simulink model "PSU"  (R2024b)
settings: Solver=VariableStepAuto  StartTime=0.0  StopTime=10.0  RelTol=1e-3
libraries: spsGroundLib x2, spsThreePhaseProgrammableVoltageSourceLib x1, spsThreePhaseBreakerLib x1, spsThreePhaseVIMeasurementLib x1, sps_lib x1
settings Model: Creator=User  LastModifiedBy=User

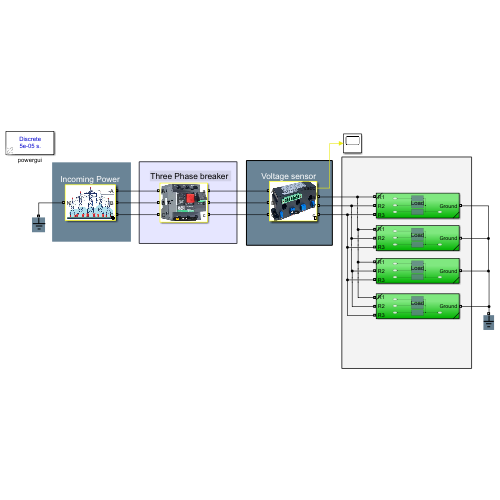
[thumbnail: Simulink's stored preview of the top-level diagram]
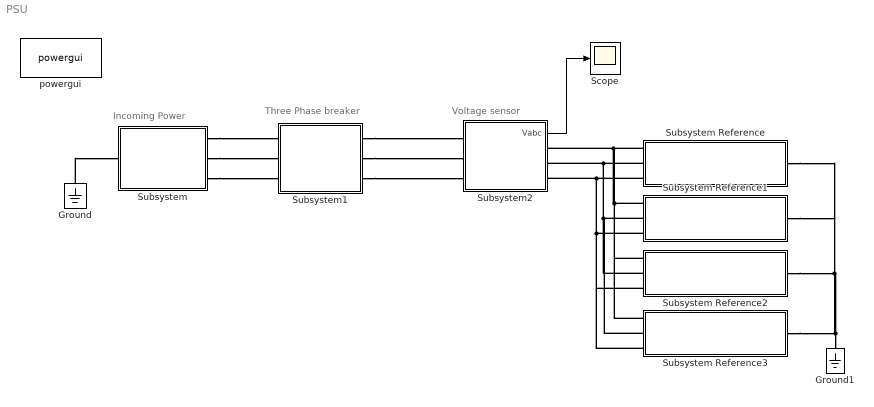
== system PSU ==
  note: Three Phase breaker
  note: Incoming Power
  note: Voltage sensor
  Ground : spsGroundLib/Ground  LConnTagsString=a
  Ground1 : spsGroundLib/Ground  LConnTagsString=a
  Scope : Scope
  Subsystem : Subsystem
      mask Display: image('Grid.png');
  Subsystem Reference{,1..3} (4 alike) : Subsystem  ReferencedSubsystem=Load
  Subsystem1 : Subsystem
      mask Display: image('Breaker.png');
  Subsystem2 : Subsystem
      mask Display: image('Voltage sensor.png');
  powergui : sps_lib/powergui  Priority=1  SimulationMode=Discrete  SampleTime=50e-6  frequency=60  Iterations=50  frequencyindice=60  Pbase=100e6  ErrMax=1e-4  UnitsV=kV  UnitsW=MW  buscounter=0  FunctionMessages=off  echomessages=off  EnableUseOfTLC=off  CurrentSourceSwitches=off  DisableSnubberDevices=off  DisableRonSwitches=off  DisableVfSwitches=off  DisplayEquations=off  AutomaticDiscreteSolvers=off  SolverType=Tustin/Backward Euler (TBE)  Interpol=off  ExternalGateDelay=off  methode=off  Ts=100  x0status=blocks  SPID=on  SwTol=0  HookPort=off  NonlinearTolerance=1e-4  nMaxIteration=100  ContinueOnMaxIteration=off  RestoreLinks=warning  ResistiveCurrentMeasurement=off  Frange=[0:2:500]  Ylog=off  Xlog=on  ShowGrid=off  save=off  variable=ZData  structure=0  ZoomFFT=off  StartTime=0.0  cycles=1  DisplayStyle=1  fundamental=60  FreqAxis=off  MaxFrequency=1000  frequencyindicesteady=1  RmsSteady=1  display=off
  wires:
  Subsystem2/1(Vabc) -> Scope/1
  connections:
  Ground/LConn1 -- Subsystem/LConn1
  Subsystem/RConn1 -- Subsystem1/LConn1
  Subsystem/RConn2 -- Subsystem1/LConn2
  Subsystem/RConn3 -- Subsystem1/LConn3
  Subsystem1/RConn1 -- Subsystem2/LConn1
  Subsystem1/RConn2 -- Subsystem2/LConn2
  Subsystem1/RConn3 -- Subsystem2/LConn3
  Subsystem Reference/LConn1 -- Subsystem Reference3/LConn1 -- Subsystem Reference2/LConn1 -- Subsystem Reference1/LConn1 -- Subsystem2/RConn1
  Subsystem Reference/LConn2 -- Subsystem Reference3/LConn2 -- Subsystem Reference2/LConn2 -- Subsystem Reference1/LConn2 -- Subsystem2/RConn2
  Subsystem Reference/LConn3 -- Subsystem Reference3/LConn3 -- Subsystem Reference2/LConn3 -- Subsystem Reference1/LConn3 -- Subsystem2/RConn3
  Subsystem Reference3/RConn1 -- Subsystem Reference1/RConn1 -- Subsystem Reference/RConn1 -- Subsystem Reference2/RConn1 -- Ground1/LConn1

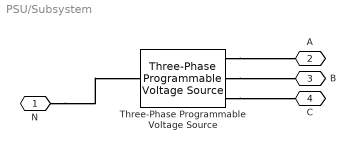
== system PSU/Subsystem ==
  Three-Phase Programmable Voltage Source : spsThreePhaseProgrammableVoltageSourceLib/Three-Phase Programmable Voltage Source  PositiveSequence="[480  0 60]"  VariationEntity=None  VariationType=Table of time-amplitude pairs  VariationTypeAlt=Step  VariationStep=0.5  VariationRate=10  VariationMagnitude=0.3  VariationFrequency=2  VariationTiming=[1 2]  VariationPhaseA=off  Amplitudes=[1 0.8 1.2 1.0]  TimeValues=[0 0.1 0.15 0.2]  HarmonicGeneration=off  HarmonicA=[3 0.2 -25 0]  HarmonicB=[2 0.15 35 2]  Timing="[0.05  3]"  BusType=swing  Pref=0  Qref=0  Qmin=-inf  Qmax=inf
  N : PMIOPort  Side=Left
  A : PMIOPort  Port=2  Side=Right
  B : PMIOPort  Port=3  Side=Right
  C : PMIOPort  Port=4  Side=Right
  connections:
  Three-Phase Programmable Voltage Source/RConn2 -- B/RConn1
  Three-Phase Programmable Voltage Source/RConn1 -- A/RConn1
  Three-Phase Programmable Voltage Source/RConn3 -- C/RConn1
  N/RConn1 -- Three-Phase Programmable Voltage Source/LConn1

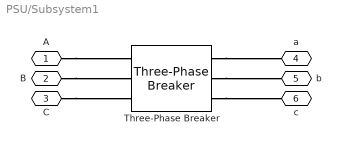
== system PSU/Subsystem1 ==
  Three-Phase Breaker : spsThreePhaseBreakerLib/Three-Phase Breaker  InitialState=closed  SwitchA=on  SwitchB=on  SwitchC=on  SwitchTimes=[2]  External=off  BreakerResistance=0.01  SnubberResistance=1e6  SnubberCapacitance=inf  Measurements=None
  A : PMIOPort  Side=Left
  B : PMIOPort  Port=2  Side=Left
  C : PMIOPort  Port=3  Side=Left
  a : PMIOPort  Port=4  Side=Right
  b : PMIOPort  Port=5  Side=Right
  c : PMIOPort  Port=6  Side=Right
  connections:
  Three-Phase Breaker/RConn1 -- a/RConn1
  Three-Phase Breaker/RConn2 -- b/RConn1
  C/RConn1 -- Three-Phase Breaker/LConn3
  A/RConn1 -- Three-Phase Breaker/LConn1
  B/RConn1 -- Three-Phase Breaker/LConn2
  Three-Phase Breaker/RConn3 -- c/RConn1

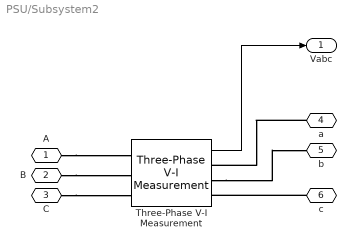
== system PSU/Subsystem2 ==
  Three-Phase V-I Measurement : spsThreePhaseVIMeasurementLib/Three-Phase V-I Measurement  VoltageMeasurement=phase-to-ground  SetLabelV=off  LabelV=Vabc  Vpu=off  VpuLL=off  CurrentMeasurement=no  SetLabelI=off  LabelI=Iabc  Ipu=off  Pbase=100e6  Vbase=500e3  OutputType=Complex  PhasorSimulation=off  PSBequivalent=0
  A : PMIOPort  Side=Left
  B : PMIOPort  Port=2  Side=Left
  C : PMIOPort  Port=3  Side=Left
  a : PMIOPort  Port=4  Side=Right
  b : PMIOPort  Port=5  Side=Right
  c : PMIOPort  Port=6  Side=Right
  Vabc : Outport
  wires:
  Three-Phase V-I Measurement/1 -> Vabc/1
  connections:
  Three-Phase V-I Measurement/RConn2 -- b/RConn1
  a/RConn1 -- Three-Phase V-I Measurement/RConn1
  A/RConn1 -- Three-Phase V-I Measurement/LConn1
  c/RConn1 -- Three-Phase V-I Measurement/RConn3
  B/RConn1 -- Three-Phase V-I Measurement/LConn2
  C/RConn1 -- Three-Phase V-I Measurement/LConn3
